simulink model "WT_ctrl"  (R2026a)
settings: Solver=FixedStepDiscrete  StopTime=inf  FixedStep=Ts
model workspace (MATLAB code in the model file):
  | % Defaults for standalone use and code generation, from HPP_parameters.
  | % In HPP.slx the Model block passes p.ctrl.wt.par as the argument "par".
  | pDefault = HPP_parameters();
  | Ts  = pDefault.ctrl.wt.Ts;    % [s] fixed sample time
  | par = pDefault.ctrl.wt.par;   % tunable parameters (model argument)
  | clear pDefault
libraries: simulink x4, sl_discontinuities x1, slpidlib x1
Description:
  | WT asset controller: IEC 61400-27-1 Type 4A control (measurement, P control type 4A, Q control with closed-loop reactive power control (MqG) and dip current injection, current limitation). Per unit on the asset rating. Parameters: model argument par (= p.ctrl.wt.par, from p.wt.iec.ctrl). Structure after the standard; details and values to be checked against it.
settings Model: ParameterArgumentNames=par  Creator=kjaer  LastModifiedBy=kjaer

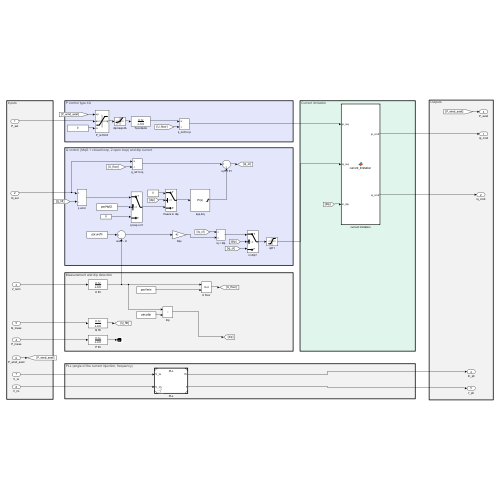
[thumbnail: Simulink's stored preview of the top-level diagram]
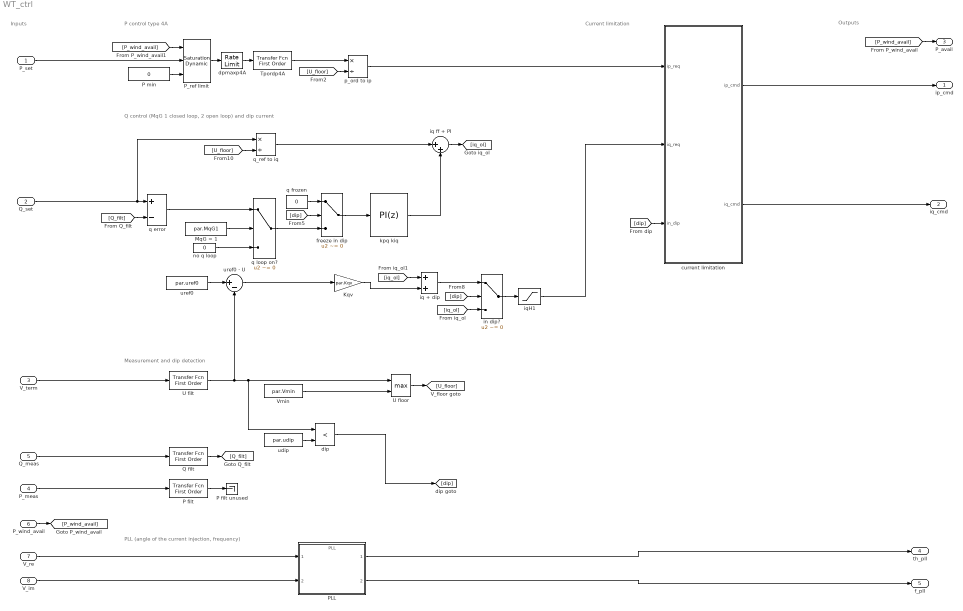
== system WT_ctrl ==
  note: Measurement and dip detection
  note: Outputs
  note: PLL (angle of the current injection, frequency)
  note: Current limitation
  note: Q control (MqG 1 closed loop, 2 open loop) and dip current
  note: P control type 4A
  note: Inputs
  P_set : Inport  OutDataTypeStr=double  PortDimensions=1  SampleTime=Ts
  Q_set : Inport  Port=2  OutDataTypeStr=double  PortDimensions=1  SampleTime=Ts
  V_term : Inport  Port=3  OutDataTypeStr=double  PortDimensions=1  SampleTime=Ts
  P_meas : Inport  Port=4  OutDataTypeStr=double  PortDimensions=1  SampleTime=Ts
  Q_meas : Inport  Port=5  OutDataTypeStr=double  PortDimensions=1  SampleTime=Ts
  P_wind_avail : Inport  Port=6  OutDataTypeStr=double  PortDimensions=1  SampleTime=Ts
  V_re : Inport  Port=7  OutDataTypeStr=double  PortDimensions=1  SampleTime=Ts
  V_im : Inport  Port=8  OutDataTypeStr=double  PortDimensions=1  SampleTime=Ts
  Kqv : Gain  Gain=par.Kqv
  MqG = 1 : Constant  Value=par.MqG1
  P filt : simulink/Discrete/Transfer Fcn First Order  PoleZ=1 - Ts/par.Tpfilt  ICPrevOutput=0  DoSatur=off
  P filt unused : Terminator
  P min : Constant  Value=0
  PLL : ModelReference  ModelNameDialog=PLL  ParameterArgumentNames=pll  ParameterArgumentValues=par.pll  UsingDefaultArgumentValue=0  SimulationMode=Normal  ModelReferenceVersion=1.1
  P_ref limit : sl_discontinuities/Saturation Dynamic  OutMin=[]  OutMax=[]  OutDataTypeStr=Inherit: Same as second input  OutDataType=fixdt(1, 16)  OutScaling=2^-10  DoSatur=off
      settings: LibrarySourceBlock=|
      | simulink/Discontinuities/Saturation
      | Dynamic
  Q filt : simulink/Discrete/Transfer Fcn First Order  PoleZ=1 - Ts/par.Tqfilt  ICPrevOutput=0  DoSatur=off
  Tpordp4A : simulink/Discrete/Transfer Fcn First Order  PoleZ=1 - Ts/par.Tpordp4A  ICPrevOutput=0  DoSatur=off
  U filt : simulink/Discrete/Transfer Fcn First Order  PoleZ=1 - Ts/par.Tufilt  ICPrevOutput=1  DoSatur=off
  U floor : MinMax  Function=max  Inputs=2
  Vmin : Constant  Value=par.Vmin
  current limitation : MATLAB Function  TreatAsAtomicUnit=on
  dip : RelationalOperator  Operator=<  OutDataTypeStr=boolean  RndMeth=Simplest  InputSameDT=off
  dpmaxp4A : RateLimiter  RisingSlewLimit=par.dpmaxp4A  FallingSlewLimit=-par.dpmaxp4A  SampleTimeMode=inherited
  freeze in dip : Switch  Criteria=u2 ~= 0  SaturateOnIntegerOverflow=off  InputSameDT=off
  in dip? : Switch  Criteria=u2 ~= 0  SaturateOnIntegerOverflow=off  InputSameDT=off
  iq + dip : Sum
  iq ff + PI : Sum  Inputs=|++
  iqH1 : Saturate  UpperLimit=par.iqH1  LowerLimit=-par.iqH1
  kpq kiq : slpidlib/PID Controller  Controller=PI  Form=Parallel  TimeDomain=Discrete-time  UseExternalTs=off  SampleTime=-1  IntegratorMethod=Forward Euler  FilterMethod=Forward Euler  ControllerParametersSource=internal  P=par.kpq  I=par.kiq  UseKiTs=off  D=0  UseExternalDerivativeSource=off  N=100  UseFilter=on  TunerSelectOption=Transfer Function Based (PID Tuner App)  InitialConditionSource=internal  InitialConditionForIntegrator=0  InitialConditionForFilter=0  DifferentiatorICPrevScaledInput=0  ExternalReset=none  TrackingMode=off  Kt=1  LimitOutput=on  SatLimitsSource=internal  UpperSaturationLimit=par.imax  LowerSaturationLimit=-par.imax  LinearizeAsGain=off  AntiWindupMode=clamping  Kb=1  LimitIntegrator=off  UpperIntegratorSaturationLimit=inf  LowerIntegratorSaturationLimit=-inf  POutMin=[]  POutMax=[]  IOutMin=[]  IOutMax=[]  DOutMin=[]  DOutMax=[]  NOutMin=[]  NOutMax=[]  SumOutMin=[]  SumOutMax=[]  SaturationOutMin=[]  SaturationOutMax=[]  PParamMin=[]  PParamMax=[]  IParamMin=[]  IParamMax=[]  DParamMin=[]  DParamMax=[]  NParamMin=[]  NParamMax=[]  KbParamMin=[]  KbParamMax=[]  KtParamMin=[]  KtParamMax=[]  KbOutMin=[]  KbOutMax=[]  KtOutMin=[]  KtOutMax=[]  IntegratorOutMin=[]  IntegratorOutMax=[]  FilterOutMin=[]  FilterOutMax=[]  SumI1OutMin=[]  SumI1OutMax=[]  SumI2OutMin=[]  SumI2OutMax=[]  SumI3OutMin=[]  SumI3OutMax=[]  SumI4OutMin=[]  SumI4OutMax=[]  SumDOutMin=[]  SumDOutMax=[]  DifferentiatorOutMin=[]  DifferentiatorOutMax=[]  FilterDiffOutCoefMin=[]  FilterDiffOutCoefMax=[]  ReciprocalOutMin=[]  ReciprocalOutMax=[]  SumDenOutMin=[]  SumDenOutMax=[]  SumNumOutMin=[]  SumNumOutMax=[]  DivideOutMin=[]  DivideOutMax=[]  UdiffTsProdOutMin=[]  UdiffTsProdOutMax=[]  NTsProdOutMin=[]  NTsProdOutMax=[]  UintegralTsProdOutMin=[]  UintegralTsProdOutMax=[]  UngainTsProdOutMin=[]  UngainTsProdOutMax=[]  ClampingZeroOutDataTypeStr=Inherit: Inherit via back propagation  ClampingZeroOutMin=[]  ClampingZeroOutMax=[]  FilterDenConstantOutDataTypeStr=Inherit: Inherit via back propagation  FilterDenConstantOutMin=[]  FilterDenConstantOutMax=[]  PCopyOutDataTypeStr=Inherit: Inherit via back propagation  PCopyOutMin=[]  PCopyOutMax=[]  NCopyOutDataTypeStr=Inherit: Inherit via back propagation  NCopyOutMin=[]  NCopyOutMax=[]  IntegratorContinuousStateAttributes=''  IntegratorStateMustResolveToSignalObject=off  IntegratorRTWStateStorageClass=Auto  FilterContinuousStateAttributes=''  FilterStateMustResolveToSignalObject=off  FilterRTWStateStorageClass=Auto  ParallelPVariant=InternalParameters  IdealPVariant=Disabled  IVariant=InternalParameters  DVariant=Disabled  IntegratorVariant=Discrete  SatVariant=Enabled  AWVariant=DiscClampingParallel  PCopyVariant=Disabled  TRVariant=Disabled  FdbkBlocksVariant=Forward  IdealPFdbkVariant=Disabled  SatFdbkVariant=Disabled  DerivativeFilterVariant=Disabled  NVariant=Disabled  NCopyVariant=Disabled_SignalSpec  FilterICVariant=Disabled  IntegratorICVariant=InternalICs  ExternalResetVariant=Disabled  TRSumVariant=Passthrough  SumFdbkVariant=Disabled  SumVariant=Sum_PI  TsampFilterVariant=InternalTs  TsampNgainVariant=Passthrough  TsampIntegralVariant=Disabled_SignalSpec  ExternalSaturationOutDataTypeStr=Inherit: Same as second input  DerivativeSourceVariant=Disabled  PreIntVariant=InternalPreInt
      settings: LibrarySourceBlock=simulink/Discrete/Discrete PID Controller
  no q loop : Constant  Value=0
  p_ord to ip : Product  Inputs=*/
  q error : Sum  Inputs=+-
  q frozen : Constant  Value=0
  q loop on? : Switch  Criteria=u2 ~= 0  SaturateOnIntegerOverflow=off  InputSameDT=off
  q_ref to iq : Product  Inputs=*/
  udip : Constant  Value=par.udip
  uref0 : Constant  Value=par.uref0
  uref0 - U : Sum  Inputs=|+-
  ip_cmd : Outport  OutDataTypeStr=double
  iq_cmd : Outport  Port=2  OutDataTypeStr=double
  P_avail : Outport  Port=3  OutDataTypeStr=double
  th_pll : Outport  Port=4  OutDataTypeStr=double
  f_pll : Outport  Port=5  OutDataTypeStr=double
  wires:
  iq + dip/1 -> in dip?/1
  Tpordp4A/1 -> p_ord to ip/1
  q_ref to iq/1 -> iq ff + PI/1
  U filt/1 -> uref0 - U/2, U floor/1, dip/1
  Vmin/1 -> U floor/2
  q error/1 -> q loop on?/1
  uref0/1 -> uref0 - U/1
  p_ord to ip/1 -> current limitation/1(ip_req)
  V_re/1 -> PLL/1
  [U_floor] -> q_ref to iq/2
  [dip] -> in dip?/2
  P_wind_avail/1 -> [P_wind_avail]
  V_term/1 -> U filt/1
  [dip] -> freeze in dip/2
  Q_set/1 -> q error/1, q_ref to iq/1
  [U_floor] -> p_ord to ip/2
  PLL/1 -> th_pll/1
  P_set/1 -> P_ref limit/2
  no q loop/1 -> q loop on?/3
  current limitation/2(iq_cmd) -> iq_cmd/1
  kpq kiq/1 -> iq ff + PI/2
  current limitation/1(ip_cmd) -> ip_cmd/1
  freeze in dip/1 -> kpq kiq/1
  dpmaxp4A/1 -> Tpordp4A/1
  udip/1 -> dip/2
  V_im/1 -> PLL/2
  U floor/1 -> [U_floor]
  MqG = 1/1 -> q loop on?/2
  q loop on?/1 -> freeze in dip/3
  q frozen/1 -> freeze in dip/1
  P min/1 -> P_ref limit/3
  P_ref limit/1 -> dpmaxp4A/1
  [P_wind_avail] -> P_avail/1
  [P_wind_avail] -> P_ref limit/1
  Q filt/1 -> [Q_filt]
  [Q_filt] -> q error/2
  dip/1 -> [dip]
  [dip] -> current limitation/3(in_dip)
  iq ff + PI/1 -> [iq_ol]
  [iq_ol] -> in dip?/3
  [iq_ol] -> iq + dip/1
  Kqv/1 -> iq + dip/2
  P filt/1 -> P filt unused/1
  PLL/2 -> f_pll/1
  P_meas/1 -> P filt/1
  Q_meas/1 -> Q filt/1
  in dip?/1 -> iqH1/1
  iqH1/1 -> current limitation/2(iq_req)
  uref0 - U/1 -> Kqv/1

== matlab function WT_ctrl/current limitation ==
  data: ip_req input; ip_cmd output; iq_req input; in_dip input; iq_cmd output; par parameter
function [ip_cmd, iq_cmd] = current_limitation(ip_req, iq_req, in_dip, par)
%#codegen
% IEC 61400-27-1 current limitation (simplified): total current <= imax;
% normal operation: active current first, reactive current gets the rest;
% during a voltage dip: reactive current first.
imax = par.imax;
if in_dip
    iq_cmd = min(max(iq_req, -imax), imax);
    ipmax  = sqrt(max(imax^2 - iq_cmd^2, 0));
    ip_cmd = min(max(ip_req, 0), ipmax);
else
    ip_cmd = min(max(ip_req, 0), imax);
    iqmax  = sqrt(max(imax^2 - ip_cmd^2, 0));
    iq_cmd = min(max(iq_req, -iqmax), iqmax);
end
end
